simulink model "GuidanceLaw"  (R2023b)
settings: Solver=ode4  StartTime=0.0  StopTime=400  FixedStep=0.05  RelTol=1e-3
values from neighbouring files (symbols this model uses):
  APCMD_TYPE : value not decoded    [apDataDictionary.sldd]
  missionRoutePlan_struct = struct(      'validWpNum_u8', uint8(5),      'missionRoute_struct', repmat(wpDefault_struct, double(maxWpNum_u8), 1))    [initMissionRoutePlan_MC.m]
  MSSN_TYPE : value not decoded    [apDataDictionary.sldd]
  setPoint_struct = struct('lat_deg_d',double(31.200000),'lon_deg_d',double(121.500000),'alt_m_f',single(100),'yaw_deg_f',single(0))    [APTest.m]
undefined symbols (not defined in the file or in its folder): apParams
libraries: simulink x13, simulink_extras x3
(part 1 of 7)
settings Model: DataDictionary=apDataDictionary.sldd  Creator=22119  LastModifiedBy=18183
settings DataIOCC: LoggingToFile=on
settings OptimizationCC: DefaultUnderspecifiedDataType=single

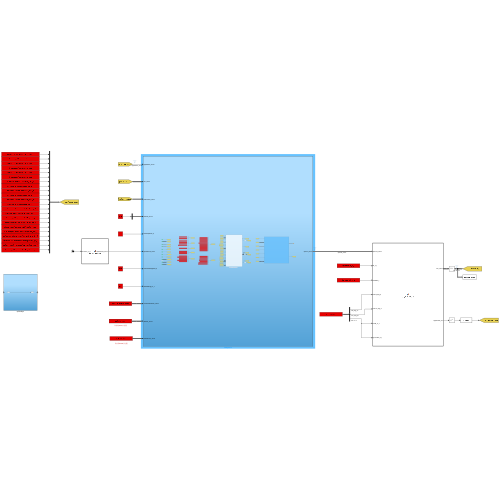
[thumbnail: Simulink's stored preview of the top-level diagram]
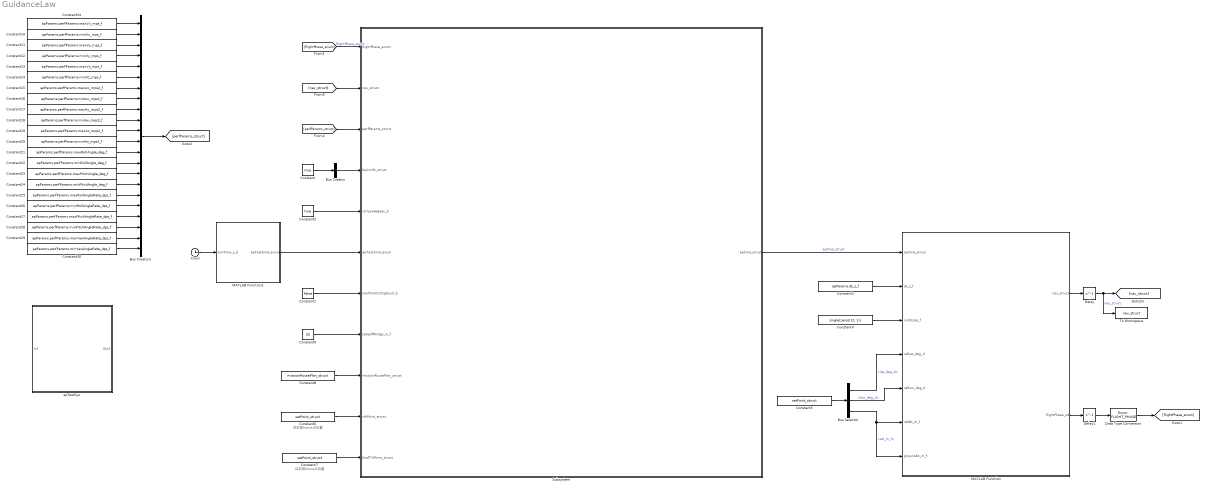
== system GuidanceLaw ==
  note: 目前是home点位置
  note: 目前用home点位置
  Bus Creator : BusCreator  Inputs=1  OutDataTypeStr=Bus: faultCaseBus
      settings: InheritFromInputs=off
  Bus Creator1 : BusCreator  Inputs=22  OutDataTypeStr=Bus: perfParamBus
      settings: InheritFromInputs=off
  Bus Selector : BusSelector  OutputSignals=lat_deg_d,lon_deg_d,alt_m_f
  Clock : Clock
  Constant : Constant  Value=true  OutDataTypeStr=boolean
  Constant1 : Constant  Value=false  OutDataTypeStr=boolean
  Constant10 : Constant  Value=apParams.perfParams.minVx_mps_f  OutDataTypeStr=single
  Constant11 : Constant  Value=apParams.perfParams.maxVy_mps_f  OutDataTypeStr=single
  Constant12 : Constant  Value=apParams.perfParams.minVy_mps_f  OutDataTypeStr=single
  Constant13 : Constant  Value=apParams.perfParams.maxVz_mps_f  OutDataTypeStr=single
  Constant14 : Constant  Value=apParams.perfParams.minVz_mps_f  OutDataTypeStr=single
  Constant15 : Constant  Value=apParams.perfParams.maxAx_mps2_f  OutDataTypeStr=single
  Constant16 : Constant  Value=apParams.perfParams.minAx_mps2_f  OutDataTypeStr=single
  Constant17 : Constant  Value=apParams.perfParams.maxAy_mps2_f  OutDataTypeStr=single
  Constant18 : Constant  Value=apParams.perfParams.minAy_mps2_f  OutDataTypeStr=single
  Constant19 : Constant  Value=apParams.perfParams.maxAz_mps2_f  OutDataTypeStr=single
  Constant2 : Constant  Value=true  OutDataTypeStr=boolean
  Constant20 : Constant  Value=apParams.perfParams.minAz_mps2_f  OutDataTypeStr=single
  Constant21 : Constant  Value=apParams.perfParams.maxRollAngle_deg_f  OutDataTypeStr=single
  Constant22 : Constant  Value=apParams.perfParams.minRollAngle_deg_f  OutDataTypeStr=single
  Constant23 : Constant  Value=apParams.perfParams.maxPitchAngle_deg_f  OutDataTypeStr=single
  Constant24 : Constant  Value=apParams.perfParams.minPitchAngle_deg_f  OutDataTypeStr=single
  Constant25 : Constant  Value=apParams.perfParams.maxRollAngleRate_dps_f  OutDataTypeStr=single
  Constant26 : Constant  Value=apParams.perfParams.minRollAngleRate_dps_f  OutDataTypeStr=single
  Constant27 : Constant  Value=apParams.perfParams.maxPitchAngleRate_dps_f  OutDataTypeStr=single
  Constant28 : Constant  Value=apParams.perfParams.minPitchAngleRate_dps_f  OutDataTypeStr=single
  Constant29 : Constant  Value=apParams.perfParams.maxYawAngleRate_dps_f  OutDataTypeStr=single
  Constant3 : Constant  Value=apParams.dt_s_f  OutDataTypeStr=single
  Constant30 : Constant  Value=apParams.perfParams.minYawAngleRate_dps_f  OutDataTypeStr=single
  Constant34 : Constant  Value=apParams.perfParams.maxVx_mps_f  OutDataTypeStr=single
  Constant4 : Constant  Value=single(zeros(12, 1))  OutDataTypeStr=single
  Constant5 : Constant  Value=setPoint_struct  OutDataTypeStr=Bus: setPointBus
  Constant6 : Constant  Value=setPoint_struct  OutDataTypeStr=Bus: setPointBus
  Constant7 : Constant  Value=setPoint_struct  OutDataTypeStr=Bus: setPointBus
  Constant8 : Constant  Value=missionRoutePlan_struct  OutDataTypeStr=Bus: missionRoutePlanBus
  Constant9 : Constant  Value=20  OutDataTypeStr=single
  Data Type Conversion : DataTypeConversion  OutDataTypeStr=Enum: FLIGHT_PHASE  SaturateOnIntegerOverflow=off  RndMeth=Floor
  Delay : Delay  DelayLength=1
  Delay1 : Delay  DelayLength=1
  MATLAB Function : MATLAB Function  TreatAsAtomicUnit=on
  MATLAB Function1 : MATLAB Function  TreatAsAtomicUnit=on
  Subsystem : Subsystem
  To Workspace : ToWorkspace  VariableName=nav_struct  SaveFormat=Timeseries  SampleTime=-1
  apTestSys : Subsystem
  wires:
  [flightPhase_enum] -> Subsystem/1(flightPhase_enum)  "flightPhase_enum"
  [perfParams_struct] -> Subsystem/3(perfParams_struct)
  Bus Creator/1 -> Subsystem/4(faultInfo_struct)
  Constant2/1 -> Subsystem/5(ctrlLawApExec_b)
  MATLAB Function1/1(apTaskCmd_enum) -> Subsystem/6(apTaskCmd_enum)
  Constant1/1 -> Subsystem/7(nonPilotCtrlSigFault_b)
  Constant9/1 -> Subsystem/8(takeoffRltHgt_m_f)
  Constant6/1 -> Subsystem/10(rthPoint_struct)
  Constant7/1 -> Subsystem/11(bwdTiltPoint_struct)
  Subsystem/1(apCmd_struct) -> MATLAB Function/1(apCmd_struct)  "apCmd_struct"
  MATLAB Function/1(nav_struct) -> Delay/1
  [nav_struct] -> Subsystem/2(nav_struct)
  Constant/1 -> Bus Creator/1
  Constant3/1 -> MATLAB Function/2(dt_s_f)
  Constant4/1 -> MATLAB Function/3(initState_f)
  Delay/1 -> To Workspace/1, [nav_struct]  "nav_struct"
  MATLAB Function/2(flightPhase_u8) -> Delay1/1
  Data Type Conversion/1 -> [flightPhase_enum]
  Delay1/1 -> Data Type Conversion/1
  Bus Creator1/1 -> [perfParams_struct]
  Constant34/1 -> Bus Creator1/1
  Constant10/1 -> Bus Creator1/2
  Constant11/1 -> Bus Creator1/3
  Constant12/1 -> Bus Creator1/4
  Constant13/1 -> Bus Creator1/5
  Constant14/1 -> Bus Creator1/6
  Constant15/1 -> Bus Creator1/7
  Constant16/1 -> Bus Creator1/8
  Constant17/1 -> Bus Creator1/9
  Constant18/1 -> Bus Creator1/10
  Constant19/1 -> Bus Creator1/11
  Constant20/1 -> Bus Creator1/12
  Constant21/1 -> Bus Creator1/13
  Constant22/1 -> Bus Creator1/14
  Constant23/1 -> Bus Creator1/15
  Constant24/1 -> Bus Creator1/16
  Constant25/1 -> Bus Creator1/17
  Constant26/1 -> Bus Creator1/18
  Constant27/1 -> Bus Creator1/19
  Constant28/1 -> Bus Creator1/20
  Clock/1 -> MATLAB Function1/1(simTime_s_d)
  Constant5/1 -> Bus Selector/1
  Bus Selector/1 -> MATLAB Function/4(refLat_deg_d)  "<lat_deg_d>"
  Bus Selector/2 -> MATLAB Function/5(refLon_deg_d)  "<lon_deg_d>"
  Bus Selector/3 -> MATLAB Function/7(groundAlt_m_f), MATLAB Function/6(refAlt_m_f)  "<alt_m_f>"
  Constant8/1 -> Subsystem/9(missionRoutePlan_struct)
  Constant29/1 -> Bus Creator1/21
  Constant30/1 -> Bus Creator1/22

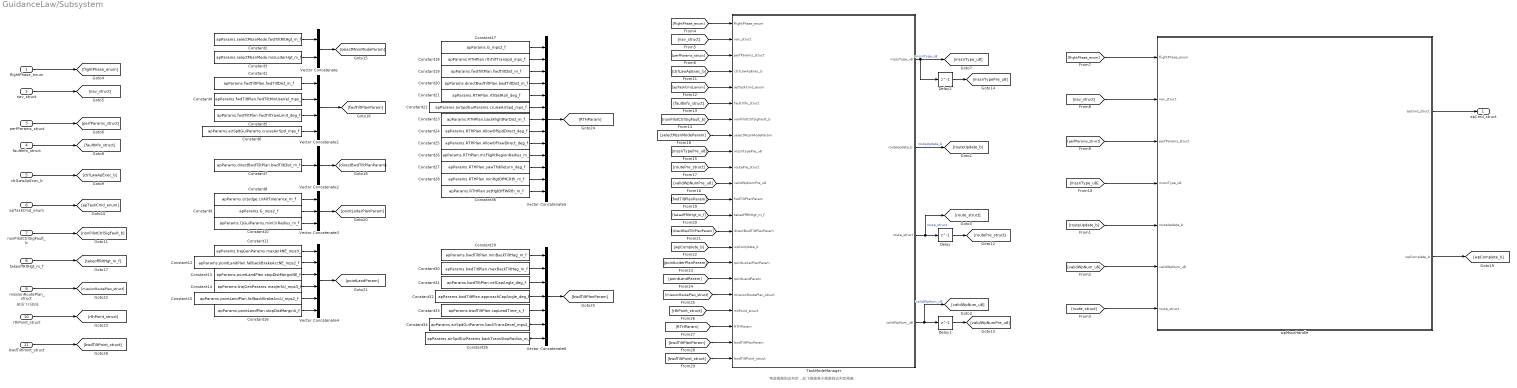
== system GuidanceLaw/Subsystem ==
  note: 航线飞行航线
  note: 考虑高度到达判定，起飞高度高于高度到达判定高度
  flightPhase_enum : Inport  OutDataTypeStr=Enum: FLIGHT_PHASE
  nav_struct : Inport  Port=2  OutDataTypeStr=Bus: apTransNavBus  BusOutputAsStruct=on
  perfParams_struct : Inport  Port=3  OutDataTypeStr=Bus: perfParamBus  BusOutputAsStruct=on
  faultInfo_struct : Inport  Port=4  OutDataTypeStr=Bus: faultCaseBus  BusOutputAsStruct=on
  ctrlLawApExec_b : Inport  Port=5  OutDataTypeStr=boolean
  apTaskCmd_enum : Inport  Port=6  OutDataTypeStr=Enum: AP_TASK_CMD
  nonPilotCtrlSigFault_b : Inport  Port=7  OutDataTypeStr=boolean
  takeoffRltHgt_m_f : Inport  Port=8  OutDataTypeStr=single
  missionRoutePlan_struct : Inport  Port=9  OutDataTypeStr=Bus: missionRoutePlanBus  BusOutputAsStruct=on
  rthPoint_struct : Inport  Port=10  OutDataTypeStr=Bus: setPointBus
  bwdTiltPoint_struct : Inport  Port=11  OutDataTypeStr=Bus: setPointBus
  Constant1 : Constant  Value=apParams.fwdTiltPlan.fwdTiltDist_m_f  OutDataTypeStr=single
  Constant10 : Constant  Value=apParams.l1GuiParams.minCirRadius_m_f  OutDataTypeStr=single
  Constant11 : Constant  Value=apParams.trajGenParams.maxJerkNE_mps3_f  OutDataTypeStr=single
  Constant12 : Constant  Value=apParams.pointLandPlan.fallbackBrakeAccNE_mps2_f  OutDataTypeStr=single
  Constant13 : Constant  Value=apParams.pointLandPlan.stopDistMarginNE_f  OutDataTypeStr=single
  Constant14 : Constant  Value=apParams.trajGenParams.maxJerkU_mps3_f  OutDataTypeStr=single
  Constant15 : Constant  Value=apParams.pointLandPlan.fallbackBrakeAccU_mps2_f  OutDataTypeStr=single
  Constant16 : Constant  Value=apParams.pointLandPlan.stopDistMarginU_f  OutDataTypeStr=single
  Constant17 : Constant  Value=apParams.G_mps2_f  OutDataTypeStr=single
  Constant18 : Constant  Value=apParams.RTHPlan.rthTiltTranSpd_mps_f  OutDataTypeStr=single
  Constant19 : Constant  Value=apParams.fwdTiltPlan.fwdTiltDist_m_f  OutDataTypeStr=single
  Constant2 : Constant  Value=apParams.selectMssnMode.fwdTiltRltHgt_m_f  OutDataTypeStr=single
  Constant20 : Constant  Value=apParams.directBwdTiltPlan.bwdTiltDist_m_f  OutDataTypeStr=single
  Constant21 : Constant  Value=apParams.RTHPlan.rthSetRoll_deg_f  OutDataTypeStr=single
  Constant22 : Constant  Value=apParams.airSpdGuiParams.cruiseAirSpd_mps_f  OutDataTypeStr=single
  Constant23 : Constant  Value=apParams.RTHPlan.backFlightFarDist_m_f  OutDataTypeStr=single
  Constant24 : Constant  Value=apParams.RTHPlan.AllowOfSpdDirect_deg_f  OutDataTypeStr=single
  Constant25 : Constant  Value=apParams.RTHPlan.AllowOfYawDirect_deg_f  OutDataTypeStr=single
  Constant26 : Constant  Value=apParams.RTHPlan.mcFlightRegionRadius_m_f  OutDataTypeStr=single
  Constant27 : Constant  Value=apParams.RTHPlan.yawThdReturn_deg_f  OutDataTypeStr=single
  Constant28 : Constant  Value=apParams.RTHPlan.minHgtOfMCRth_m_f  OutDataTypeStr=single
  Constant29 : Constant  Value=apParams.bwdTiltPlan.minBackTiltHag_m_f  OutDataTypeStr=single
  Constant3 : Constant  Value=apParams.selectMssnMode.minLoiterHgt_m_f  OutDataTypeStr=single
  Constant30 : Constant  Value=apParams.bwdTiltPlan.maxBackTiltHag_m_f  OutDataTypeStr=single
  Constant31 : Constant  Value=apParams.bwdTiltPlan.velCapAngle_deg_f  OutDataTypeStr=single
  Constant32 : Constant  Value=apParams.bwdTiltPlan.approachCapAngle_deg_f  OutDataTypeStr=single
  Constant33 : Constant  Value=apParams.bwdTiltPlan.capLeadTime_s_f  OutDataTypeStr=single
  Constant34 : Constant  Value=apParams.airSpdGuiParams.backTransDecel_mps2_f  OutDataTypeStr=single
  Constant35 : Constant  Value=apParams.airSpdGuiParams.backTransStopRadius_m_f  OutDataTypeStr=single
  Constant36 : Constant  Value=apParams.RTHPlan.setHgtOfFWRth_m_f  OutDataTypeStr=single
  Constant4 : Constant  Value=apParams.fwdTiltPlan.fwdTiltMinUseVel_mps_f  OutDataTypeStr=single
  Constant5 : Constant  Value=apParams.fwdTiltPlan.fwdTiltYawLimit_deg_f  OutDataTypeStr=single
  Constant6 : Constant  Value=apParams.airSpdGuiParams.cruiseAirSpd_mps_f  OutDataTypeStr=single
  Constant7 : Constant  Value=apParams.directBwdTiltPlan.bwdTiltDist_m_f  OutDataTypeStr=single
  Constant8 : Constant  Value=apParams.cirJudge.cirAltTolerance_m_f  OutDataTypeStr=single
  Constant9 : Constant  Value=apParams.G_mps2_f  OutDataTypeStr=single
  Delay : Delay  DelayLength=1  InitialCondition=apParams.defaultRoute_struct
  Delay1 : Delay  DelayLength=1  InitialCondition=uint8(0)
  Delay2 : Delay  DelayLength=1  InitialCondition=MSSN_TYPE.IDLE
  TaskModeManager : Stateflow chart  TreatAsAtomicUnit=on
  Vector Concatenate : Concatenate
  Vector Concatenate1 : Concatenate  NumInputs=4
  Vector Concatenate2 : Concatenate  NumInputs=1
  Vector Concatenate3 : Concatenate  NumInputs=3
  Vector Concatenate4 : Concatenate  NumInputs=6
  Vector Concatenate5 : Concatenate  NumInputs=13
  Vector Concatenate6 : Concatenate  NumInputs=7
  wpMssnHandle : Subsystem
  apCmd_struct : Outport  OutDataTypeStr=Bus: apCmdBus
  wires:
  TaskModeManager/2(routeUpdate_b) -> [routeUpdate_b]  "routeUpdate_b"
  [perfParams_struct] -> wpMssnHandle/3(perfParams_struct)
  Constant30/1 -> Vector Concatenate6/2
  Constant19/1 -> Vector Concatenate5/3
  Vector Concatenate1/1 -> [fwdTiltPlanParam]
  [flightPhase_enum] -> wpMssnHandle/1(flightPhase_enum)
  [ctrlLawApExec_b] -> TaskModeManager/4(ctrlLawApExec_b)
  Constant17/1 -> Vector Concatenate5/1
  [nav_struct] -> TaskModeManager/2(nav_struct)
  Delay2/1 -> [mssnTypePre_u8]
  Vector Concatenate4/1 -> [pointLandParam]
  Constant32/1 -> Vector Concatenate6/4
  [routeUpdate_b] -> wpMssnHandle/5(routeUpdate_b)
  [rthPoint_struct] -> TaskModeManager/19(rthPoint_struct)
  [nonPilotCtrlSigFault_b] -> TaskModeManager/7(nonPilotCtrlSigFault_b)
  [mssnType_u8] -> wpMssnHandle/4(mssnType_u8)
  flightPhase_enum/1 -> [flightPhase_enum]
  [pointLandParam] -> TaskModeManager/17(pointLandParam)
  Constant25/1 -> Vector Concatenate5/9
  faultInfo_struct/1 -> [faultInfo_struct]
  [takeoffRltHgt_m_f] -> TaskModeManager/13(takeoffRltHgt_m_f)
  [validWpNumPre_u8] -> TaskModeManager/11(validWpNumPre_u8)
  Vector Concatenate6/1 -> [bwdTiltPlanParam]
  [faultInfo_struct] -> TaskModeManager/6(faultInfo_struct)
  perfParams_struct/1 -> [perfParams_struct]
  Constant21/1 -> Vector Concatenate5/5
  Constant29/1 -> Vector Concatenate6/1
  ctrlLawApExec_b/1 -> [ctrlLawApExec_b]
  [nav_struct] -> wpMssnHandle/2(nav_struct)
  Vector Concatenate5/1 -> [RTHParam]
  [routePre_struct] -> TaskModeManager/10(routePre_struct)
  Constant33/1 -> Vector Concatenate6/5
  Constant18/1 -> Vector Concatenate5/2
  Constant20/1 -> Vector Concatenate5/4
  [missionRoutePlan_struct] -> TaskModeManager/18(missionRoutePlan_struct)
  Constant22/1 -> Vector Concatenate5/6
  TaskModeManager/1(mssnType_u8) -> Delay2/1, [mssnType_u8]  "mssnType_u8"
  [fwdTiltPlanParam] -> TaskModeManager/12(fwdTiltPlanParam)
  [bwdTiltPoint_struct] -> TaskModeManager/22(bwdTiltPoint_struct)
  Constant11/1 -> Vector Concatenate4/1
  apTaskCmd_enum/1 -> [apTaskCmd_enum]
  [flightPhase_enum] -> TaskModeManager/1(flightPhase_enum)
  Constant4/1 -> Vector Concatenate1/2
  [pointLoiterPlanParam] -> TaskModeManager/16(pointLoiterPlanParam)
  Constant1/1 -> Vector Concatenate1/1
  [RTHParam] -> TaskModeManager/20(RTHParam)
  [perfParams_struct] -> TaskModeManager/3(perfParams_struct)
  TaskModeManager/3(route_struct) -> [route_struct], Delay/1  "route_struct"
  Constant12/1 -> Vector Concatenate4/2
  [wpComplete_b] -> TaskModeManager/15(wpComplete_b)
  Constant15/1 -> Vector Concatenate4/5
  Vector Concatenate3/1 -> [pointLoiterPlanParam]
  [directBwdTiltPlanParam] -> TaskModeManager/14(directBwdTiltPlanParam)
  Constant23/1 -> Vector Concatenate5/7
  Constant27/1 -> Vector Concatenate5/11
  Constant14/1 -> Vector Concatenate4/4
  Constant8/1 -> Vector Concatenate3/1
  Vector Concatenate2/1 -> [directBwdTiltPlanParam]
  Constant3/1 -> Vector Concatenate/2
  [route_struct] -> wpMssnHandle/7(route_struct)
  Delay1/1 -> [validWpNumPre_u8]
  [apTaskCmd_enum] -> TaskModeManager/5(apTaskCmd_enum)
  nonPilotCtrlSigFault_b/1 -> [nonPilotCtrlSigFault_b]
  wpMssnHandle/1(apCmd_struct) -> apCmd_struct/1
  Constant2/1 -> Vector Concatenate/1
  [validWpNum_u8] -> wpMssnHandle/6(validWpNum_u8)
  Constant28/1 -> Vector Concatenate5/12
  Constant26/1 -> Vector Concatenate5/10
  Constant13/1 -> Vector Concatenate4/3
  Constant10/1 -> Vector Concatenate3/3
  Constant24/1 -> Vector Concatenate5/8
  rthPoint_struct/1 -> [rthPoint_struct]
  TaskModeManager/4(validWpNum_u8) -> [validWpNum_u8], Delay1/1  "validWpNum_u8"
  nav_struct/1 -> [nav_struct]
  Constant6/1 -> Vector Concatenate1/4
  Vector Concatenate/1 -> [selectMssnModeParam]
  Constant5/1 -> Vector Concatenate1/3
  Constant31/1 -> Vector Concatenate6/3
  [selectMssnModeParam] -> TaskModeManager/8(selectMssnModeParam)
  bwdTiltPoint_struct/1 -> [bwdTiltPoint_struct]
  missionRoutePlan_struct/1 -> [missionRoutePlan_struct]
  [mssnTypePre_u8] -> TaskModeManager/9(mssnTypePre_u8)
  takeoffRltHgt_m_f/1 -> [takeoffRltHgt_m_f]
  [bwdTiltPlanParam] -> TaskModeManager/21(bwdTiltPlanParam)
  Constant16/1 -> Vector Concatenate4/6
  Constant7/1 -> Vector Concatenate2/1
  Constant34/1 -> Vector Concatenate6/6
  Delay/1 -> [routePre_struct]
  Constant9/1 -> Vector Concatenate3/2
  wpMssnHandle/2(wpComplete_b) -> [wpComplete_b]
  Constant35/1 -> Vector Concatenate6/7
  Constant36/1 -> Vector Concatenate5/13

== system GuidanceLaw/apTestSys ==
  In1 : Inport
  Out1 : Outport
  wires:
  In1/1 -> Out1/1

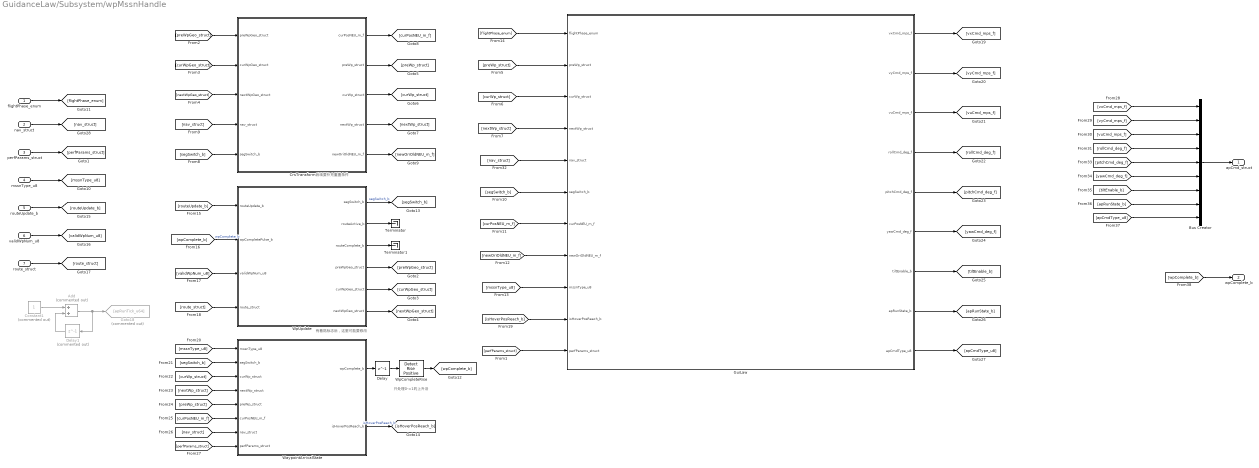
== system GuidanceLaw/Subsystem/wpMssnHandle ==
  note: 后续要补充重置条件
  note: 只处理0->1的上升沿
  note: 有着陆标志后，这里可能要修改
  flightPhase_enum : Inport
  nav_struct : Inport  Port=2
  perfParams_struct : Inport  Port=3
  mssnType_u8 : Inport  Port=4
  routeUpdate_b : Inport  Port=5
  validWpNum_u8 : Inport  Port=6
  route_struct : Inport  Port=7  PortDimensions=[30,1]  BusOutputAsStruct=on
  Add : Sum  Commented=on  OutDataTypeStr=uint64  AccumDataTypeStr=uint64
  Bus Creator : BusCreator  Inputs=9  OutDataTypeStr=Bus: apCmdBus
      settings: InheritFromInputs=off
  Constant1 : Constant  Commented=on  OutDataTypeStr=uint64
  CrsTransform : Subsystem
  Delay : Delay  DelayLength=1  InitialCondition=false
  Delay1 : Delay  Commented=on  DelayLength=1  InitialCondition=uint64(0)
  Goto18 : Goto  Commented=on  GotoTag=apRunTick_u64
  GuiLaw : Subsystem
  Terminator : Terminator
  Terminator1 : Terminator
  WaypointArrivalState : Subsystem
  WpCompleteRise : simulink/Logic and Bit Operations/Detect Rise Positive  vinit=0  OutDataTypeStr=boolean
  WpUpdate : Subsystem
  apCmd_struct : Outport  OutDataTypeStr=Bus: apCmdBus
  wpComplete_b : Outport  Port=2
  wires:
  [preWp_struct] -> WaypointArrivalState/5(preWp_struct)
  mssnType_u8/1 -> [mssnType_u8]
  GuiLaw/6(yawCmd_deg_f) -> [yawCmd_deg_f]
  WpUpdate/6(nextWpGeo_struct) -> [nextWpGeo_struct]
  [newOriOldNEU_m_f] -> GuiLaw/8(newOriOldNEU_m_f)
  [segSwitch_b] -> WaypointArrivalState/2(segSwitch_b)
  WpUpdate/5(curWpGeo_struct) -> [curWpGeo_struct]
  [isHoverPosReach_b] -> GuiLaw/10(isHoverPosReach_b)
  WpUpdate/4(preWpGeo_struct) -> [preWpGeo_struct]
  GuiLaw/7(tiltEnable_b) -> [tiltEnable_b]
  WaypointArrivalState/1(wpComplete_b) -> Delay/1
  [flightPhase_enum] -> GuiLaw/1(flightPhase_enum)
  [segSwitch_b] -> GuiLaw/6(segSwitch_b)
  [segSwitch_b] -> CrsTransform/5(segSwitch_b)
  WaypointArrivalState/2(isHoverPosReach_b) -> [isHoverPosReach_b]  "isHoverPosReach_b"
  nav_struct/1 -> [nav_struct]
  WpUpdate/1(segSwitch_b) -> [segSwitch_b]  "segSwitch_b"
  WpUpdate/2(routeActive_b) -> Terminator/1
  [curWp_struct] -> WaypointArrivalState/3(curWp_struct)
  GuiLaw/3(vuCmd_mps_f) -> [vuCmd_mps_f]
  Delay/1 -> WpCompleteRise/1
  [mssnType_u8] -> GuiLaw/9(mssnType_u8)
  [nextWp_struct] -> WaypointArrivalState/4(nextWp_struct)
  CrsTransform/5(newOriOldNEU_m_f) -> [newOriOldNEU_m_f]
  CrsTransform/1(curPosNEU_m_f) -> [curPosNEU_m_f]
  GuiLaw/4(rollCmd_deg_f) -> [rollCmd_deg_f]
  Add/1 -> Delay1/1, Goto18/1
  [preWp_struct] -> GuiLaw/2(preWp_struct)
  [route_struct] -> WpUpdate/4(route_struct)
  Delay1/1 -> Add/2
  [mssnType_u8] -> WaypointArrivalState/1(mssnType_u8)
  [nav_struct] -> WaypointArrivalState/7(nav_struct)
  [perfParams_struct] -> GuiLaw/11(perfParams_struct)
  validWpNum_u8/1 -> [validWpNum_u8]
  [curWpGeo_struct] -> CrsTransform/2(curWpGeo_struct)
  CrsTransform/4(nextWp_struct) -> [nextWp_struct]
  route_struct/1 -> [route_struct]
  [curPosNEU_m_f] -> WaypointArrivalState/6(curPosNEU_m_f)
  GuiLaw/9(apCmdType_u8) -> [apCmdType_u8]
  WpUpdate/3(routeComplete_b) -> Terminator1/1
  flightPhase_enum/1 -> [flightPhase_enum]
  GuiLaw/5(pitchCmd_deg_f) -> [pitchCmd_deg_f]
  [curPosNEU_m_f] -> GuiLaw/7(curPosNEU_m_f)
  Constant1/1 -> Add/1
  GuiLaw/8(apRunState_b) -> [apRunState_b]
  GuiLaw/2(vyCmd_mps_f) -> [vyCmd_mps_f]
  [perfParams_struct] -> WaypointArrivalState/8(perfParams_struct)
  perfParams_struct/1 -> [perfParams_struct]
  [routeUpdate_b] -> WpUpdate/1(routeUpdate_b)
  CrsTransform/3(curWp_struct) -> [curWp_struct]
  [nextWpGeo_struct] -> CrsTransform/3(nextWpGeo_struct)
  routeUpdate_b/1 -> [routeUpdate_b]
  [nav_struct] -> CrsTransform/4(nav_struct)
  CrsTransform/2(preWp_struct) -> [preWp_struct]
  [preWpGeo_struct] -> CrsTransform/1(preWpGeo_struct)
  [wpComplete_b] -> WpUpdate/2(wpCompletePulse_b)  "wpComplete_b"
  [nav_struct] -> GuiLaw/5(nav_struct)
  [curWp_struct] -> GuiLaw/3(curWp_struct)
  [nextWp_struct] -> GuiLaw/4(nextWp_struct)
  [validWpNum_u8] -> WpUpdate/3(validWpNum_u8)
  GuiLaw/1(vxCmd_mps_f) -> [vxCmd_mps_f]
  [vxCmd_mps_f] -> Bus Creator/1
  [vyCmd_mps_f] -> Bus Creator/2
  [vuCmd_mps_f] -> Bus Creator/3
  [rollCmd_deg_f] -> Bus Creator/4
  [pitchCmd_deg_f] -> Bus Creator/5
  [yawCmd_deg_f] -> Bus Creator/6
  [tiltEnable_b] -> Bus Creator/7
  [apRunState_b] -> Bus Creator/8
  [apCmdType_u8] -> Bus Creator/9
  Bus Creator/1 -> apCmd_struct/1
  [wpComplete_b] -> wpComplete_b/1
  WpCompleteRise/1 -> [wpComplete_b]

== system GuidanceLaw/Subsystem/wpMssnHandle/CrsTransform ==
  preWpGeo_struct : Inport
  curWpGeo_struct : Inport  Port=2
  nextWpGeo_struct : Inport  Port=3
  nav_struct : Inport  Port=4
  segSwitch_b : Inport  Port=5
  Bus Creator : BusCreator  Inputs=11  OutDataTypeStr=Bus: localNEUWpBus
      settings: InheritFromInputs=off
  Bus Creator1 : BusCreator  Inputs=11  OutDataTypeStr=Bus: localNEUWpBus
      settings: InheritFromInputs=off
  Bus Creator2 : BusCreator  Inputs=11  OutDataTypeStr=Bus: localNEUWpBus
      settings: InheritFromInputs=off
  Bus Selector : BusSelector  OutputSignals=wpType_u8,spd_mps_f,radius_m_f,fastWp_b,yawType_u8,yaw_deg_f,timeOrCount_u16,arrivalCond_u8
  Bus Selector1 : BusSelector  OutputSignals=wpType_u8,spd_mps_f,radius_m_f,fastWp_b,yawType_u8,yaw_deg_f,timeOrCount_u16,arrivalCond_u8
  Bus Selector2 : BusSelector  OutputSignals=wpType_u8,spd_mps_f,radius_m_f,fastWp_b,yawType_u8,yaw_deg_f,timeOrCount_u16,arrivalCond_u8
  Demux : Demux  Outputs=3
  Demux1 : Demux  Outputs=3
  Demux2 : Demux  Outputs=3
  geoToLocalNEU : MATLAB Function  TreatAsAtomicUnit=on
  curPosNEU_m_f : Outport
  preWp_struct : Outport  Port=2
  curWp_struct : Outport  Port=3
  nextWp_struct : Outport  Port=4
  newOriOldNEU_m_f : Outport  Port=5
  wires:
  preWpGeo_struct/1 -> [preWpGeo_struct]
  curWpGeo_struct/1 -> [curWpGeo_struct]
  nextWpGeo_struct/1 -> [nextWpGeo_struct]
  [preWpGeo_struct] -> geoToLocalNEU/2(preWpGeo_struct)
  [curWpGeo_struct] -> geoToLocalNEU/3(curWpGeo_struct)
  [nextWpGeo_struct] -> geoToLocalNEU/4(nextWpGeo_struct)
  nav_struct/1 -> [nav_struct]
  [nav_struct] -> geoToLocalNEU/1(curGeo_struct)
  [segSwitch_b] -> geoToLocalNEU/5(segSwitch_b)
  segSwitch_b/1 -> [segSwitch_b]
  geoToLocalNEU/1(curPosNEU_m_f) -> curPosNEU_m_f/1
  geoToLocalNEU/5(newOriOldNEU_m_f) -> newOriOldNEU_m_f/1
  [preWpGeo_struct] -> Bus Selector/1
  Bus Selector/1 -> Bus Creator/1  "<wpType_u8>"
  Bus Selector/2 -> Bus Creator/5  "<spd_mps_f>"
  Bus Selector/3 -> Bus Creator/6  "<radius_m_f>"
  Bus Selector/4 -> Bus Creator/7  "<fastWp_b>"
  Bus Selector/5 -> Bus Creator/8  "<yawType_u8>"
  Bus Selector/6 -> Bus Creator/9  "<yaw_deg_f>"
  geoToLocalNEU/2(preWpNEU_m_f) -> [preWpNEU_m_f]
  geoToLocalNEU/3(curWpNEU_m_f) -> [curWpNEU_m_f]
  geoToLocalNEU/4(nextWpNEU_m_f) -> [nextWpNEU_m_f]
  Bus Creator/1 -> preWp_struct/1
  Demux/1 -> Bus Creator/2
  Demux/2 -> Bus Creator/3
  Demux/3 -> Bus Creator/4
  [preWpNEU_m_f] -> Demux/1
  Demux1/2 -> Bus Creator1/3
  Demux1/1 -> Bus Creator1/2
  Bus Creator1/1 -> curWp_struct/1
  [curWpGeo_struct] -> Bus Selector1/1
  Bus Selector1/2 -> Bus Creator1/5  "<spd_mps_f>"
  Bus Selector1/3 -> Bus Creator1/6  "<radius_m_f>"
  Bus Selector1/6 -> Bus Creator1/9  "<yaw_deg_f>"
  Bus Selector1/5 -> Bus Creator1/8  "<yawType_u8>"
  Bus Selector1/4 -> Bus Creator1/7  "<fastWp_b>"
  Bus Selector1/1 -> Bus Creator1/1  "<wpType_u8>"
  Demux1/3 -> Bus Creator1/4
  [curWpNEU_m_f] -> Demux1/1
  Bus Selector2/1 -> Bus Creator2/1  "<wpType_u8>"
  Demux2/3 -> Bus Creator2/4
  [nextWpNEU_m_f] -> Demux2/1
  Bus Selector2/4 -> Bus Creator2/7  "<fastWp_b>"
  Bus Selector2/6 -> Bus Creator2/9  "<yaw_deg_f>"
  Bus Selector2/3 -> Bus Creator2/6  "<radius_m_f>"
  Bus Selector2/2 -> Bus Creator2/5  "<spd_mps_f>"
  Demux2/2 -> Bus Creator2/3
  Bus Selector2/5 -> Bus Creator2/8  "<yawType_u8>"
  [nextWpGeo_struct] -> Bus Selector2/1
  Demux2/1 -> Bus Creator2/2
  Bus Creator2/1 -> nextWp_struct/1
  Bus Selector/7 -> Bus Creator/10  "<timeOrCount_u16>"
  Bus Selector/8 -> Bus Creator/11  "<arrivalCond_u8>"
  Bus Selector1/7 -> Bus Creator1/10  "<timeOrCount_u16>"
  Bus Selector1/8 -> Bus Creator1/11  "<arrivalCond_u8>"
  Bus Selector2/7 -> Bus Creator2/10  "<timeOrCount_u16>"
  Bus Selector2/8 -> Bus Creator2/11  "<arrivalCond_u8>"

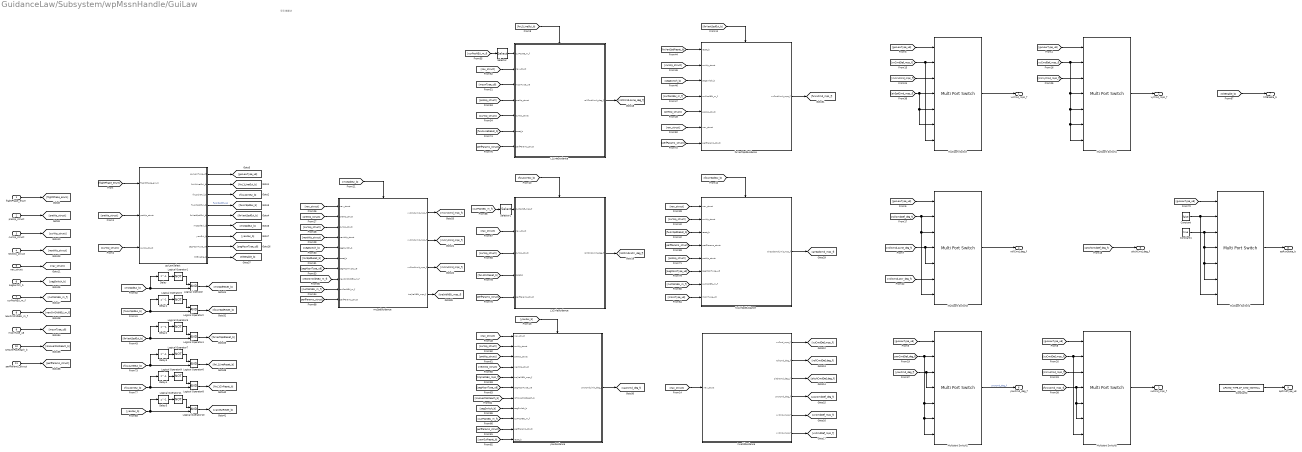
== system GuidanceLaw/Subsystem/wpMssnHandle/GuiLaw ==
  note: 导引律算法
  flightPhase_enum : Inport
  preWp_struct : Inport  Port=2
  curWp_struct : Inport  Port=3
  nextWp_struct : Inport  Port=4
  nav_struct : Inport  Port=5
  segSwitch_b : Inport  Port=6
  curPosNEU_m_f : Inport  Port=7
  newOriOldNEU_m_f : Inport  Port=8
  mssnType_u8 : Inport  Port=9
  isHoverPosReach_b : Inport  Port=10
  perfParams_struct : Inport  Port=11
  Constant : Constant  Value=false  OutDataTypeStr=boolean
  Constant1 : Constant  Value=true  OutDataTypeStr=boolean
  Constant2 : Constant  Value=APCMD_TYPE.AP_CMD_NORMAL  VectorParams1D=off  OutDataTypeStr=Enum: APCMD_TYPE
  Delay{,1..5} (6 alike) : Delay  DelayLength=1  InitialCondition=false
  L1CirleGuidance : Subsystem
  L1LineGuidance : Subsystem
  Logical Operator{,2,4,6,8,10} (6 alike) : Logic  AllPortsSameDT=off  OutDataTypeStr=boolean
  Logical Operator{1,3,5,7,9,11} (6 alike) : Logic  Operator=NOT  AllPortsSameDT=off  OutDataTypeStr=boolean
  Multiport Switch{,1..5} (6 alike) : MultiPortSwitch  DataPortOrder=Zero-based contiguous  Inputs=5  DataPortForDefault=Additional data port  DiagnosticForDefault=None  zeroidx=on  SaturateOnIntegerOverflow=off  InputSameDT=off
  Selector : Selector  InputPortWidth=3  IndexOptions=Index vector (dialog)  Indices=[1 2]  OutputSizes=1
  Selector1 : Selector  InputPortWidth=3  IndexOptions=Index vector (dialog)  Indices=[1 2]  OutputSizes=1
  fwAirSpdGuidance : Subsystem
  fwVertSpdGuidance : Subsystem
  guiLawSelect : Subsystem
  invaildGuidance : Subsystem
  mcSpdGuidance : Subsystem
  yawGuidance : Subsystem
  vxCmd_mps_f : Outport
  vyCmd_mps_f : Outport  Port=2
  vuCmd_mps_f : Outport  Port=3
  rollCmd_deg_f : Outport  Port=4
  pitchCmd_deg_f : Outport  Port=5
  yawCmd_deg_f : Outport  Port=6
  tiltEnable_b : Outport  Port=7
  apRunState_b : Outport  Port=8
  apCmdType_u8 : Outport  Port=9
  wires:
  [preWp_struct] -> fwVertSpdGuidance/5(preWp_struct)
  [mcSpdGui_b] -> mcSpdGuidance/Enable
  [yawCmd_deg_f] -> Multiport Switch2/4, Multiport Switch2/3
  [segMssnType_u8] -> mcSpdGuidance/7(segMssnType_u8)
  [preWp_struct] -> L1LineGuidance/4(preWp_struct)
  [rollCmdL1Line_deg_f] -> Multiport Switch3/5, Multiport Switch3/4
  guiLawSelect/7(yawGui_b) -> [yawGui_b]
  [segSwitch_b] -> fwVertSpdGuidance/3(segSwitch_b)
  [curPosNEU_m_f] -> Selector/1
  Logical Operator/1 -> [mcSpdReset_b]
  [nav_struct] -> yawGuidance/1(nav_struct)
  [curPosNEU_m_f] -> fwVertSpdGuidance/4(curPosNEU_m_f)
  [segSwitch_b] -> yawGuidance/8(segSwitch_b)
  [fwL1CirGui_b] -> L1CirleGuidance/Enable
  [rollCmdDef_deg_f] -> Multiport Switch3/3, Multiport Switch3/7, Multiport Switch3/2
  [curPosNEU_m_f] -> Selector1/1
  [fwAirSpdGui_b] -> fwAirSpdGuidance/Enable
  [guiLawType_u8] -> Multiport Switch2/1
  [preWp_struct] -> guiLawSelect/2(preWp_struct)
  [airSpdCmd_mps_f] -> Multiport Switch/6, Multiport Switch/5, Multiport Switch/4
  guiLawSelect/1(guiLawType_u8) -> [guiLawType_u8]
  [fwVertSpdGui_b] -> Delay2/1, Logical Operator4/2
  [curWp_struct] -> fwAirSpdGuidance/2(curWp_struct)
  Delay2/1 -> Logical Operator5/1
  mcSpdGuidance/1(vxCmdLimit_mps_f) -> [mcVxCmd_mps_f]
  Multiport Switch3/1 -> rollCmd_deg_f/1
  mcSpdGuidance/4(trajVelNEU_mps_f) -> [trajVelNEU_mps_f]
  [vxCmdDef_mps_f] -> Multiport Switch/7, Multiport Switch/2
  [guiLawType_u8] -> Multiport Switch3/1
  [guiLawType_u8] -> Multiport Switch/1
  [guiLawType_u8] -> Multiport Switch1/1
  [flightPhase_enum] -> guiLawSelect/1(flightPhase_enum)
  guiLawSelect/4(fwAirSpdGui_b) -> [fwAirSpdGui_b]  "fwAirSpdGui_b"
  [mcSpdGui_b] -> Delay/1, Logical Operator/2
  segSwitch_b/1 -> [segSwitch_b]
  curWp_struct/1 -> [curWp_struct]
  Multiport Switch5/1 -> vuCmd_mps_f/1
  [trajVelNEU_mps_f] -> yawGuidance/5(trajVelNEU_mps_f)
  mssnType_u8/1 -> [mssnType_u8]
  Logical Operator5/1 -> Logical Operator4/1
  [nav_struct] -> fwAirSpdGuidance/1(nav_struct)
  guiLawSelect/5(fwVertSpdGui_b) -> [fwVertSpdGui_b]
  [nav_struct] -> fwVertSpdGuidance/6(nav_struct)
  Delay1/1 -> Logical Operator3/1
  [segMssnType_u8] -> yawGuidance/6(segMssnType_u8)
  [fwAirSpdReset_b] -> fwAirSpdGuidance/3(reset_b)
  [nav_struct] -> L1LineGuidance/2(nav_struct)
  [fwVertSpdGui_b] -> fwVertSpdGuidance/Enable
  [mcVuCmd_mps_f] -> Multiport Switch5/3
  [mssnType_u8] -> L1LineGuidance/3(mssnType_u8)
  [mcVxCmd_mps_f] -> Multiport Switch/3
  yawGuidance/1(yawCmdLimit_deg_f) -> [yawCmd_deg_f]
  [isHoverPosReach_b] -> yawGuidance/7(isHoverPosReach_b)
  [curWp_struct] -> L1CirleGuidance/3(curWp_struct)
  guiLawSelect/3(fwL1CirGui_b) -> [fwL1CirGui_b]
  [newOriOldNEU_m_f] -> mcSpdGuidance/8(newOriOldNEU_m_f)
  invaildGuidance/1(vuCmd_mps_f) -> [vuCmdDef_mps_f]
  guiLawSelect/6(mcSpdGui_b) -> [mcSpdGui_b]
  [curWp_struct] -> yawGuidance/2(curWp_struct)
  [nextWp_struct] -> yawGuidance/4(nextWp_struct)
  [curWp_struct] -> fwVertSpdGuidance/2(curWp_struct)
  [preWp_struct] -> yawGuidance/3(preWp_struct)
  [rollCmdL1Cir_deg_f] -> Multiport Switch3/6
  Selector1/1 -> L1CirleGuidance/1(curPosNE_mps_f)
  [fwL1LineGui_b] -> L1LineGuidance/Enable
  [curWp_struct] -> guiLawSelect/3(curWp_struct)
  isHoverPosReach_b/1 -> [isHoverPosReach_b]
  [mcVyCmd_mps_f] -> Multiport Switch1/3
  guiLawSelect/2(fwL1LineGui_b) -> [fwL1LineGui_b]
  Selector/1 -> L1LineGuidance/1(curPosNE_m_f)
  preWp_struct/1 -> [preWp_struct]
  [nav_struct] -> L1CirleGuidance/2(nav_struct)
  invaildGuidance/4(yawCmd_deg_f) -> [yawCmdDef_deg_f]
  [yawGui_b] -> yawGuidance/Enable
  L1CirleGuidance/1(rollCmdLimit_deg_f) -> [rollCmdL1Cir_deg_f]
  [guiLawType_u8] -> Multiport Switch5/1
  nav_struct/1 -> [nav_struct]
  invaildGuidance/6(vxCmd_mps_f) -> [vxCmdDef_mps_f]
  [vyCmdDef_mps_f] -> Multiport Switch1/4, Multiport Switch1/6, Multiport Switch1/7, Multiport Switch1/5, Multiport Switch1/2
  Logical Operator4/1 -> [fwVertSpdReset_b]
  Logical Operator3/1 -> Logical Operator2/1
  [yawCmdDef_deg_f] -> Multiport Switch2/5, Multiport Switch2/6, Multiport Switch2/7, Multiport Switch2/2
  [nav_struct] -> invaildGuidance/1(nav_struct)
  mcSpdGuidance/3(vuCmdLimit_mps_f) -> [mcVuCmd_mps_f]
  Multiport Switch/1 -> vxCmd_mps_f/1
  fwAirSpdGuidance/1(airSpdCmdLimit_mps_f) -> [airSpdCmd_mps_f]
  Multiport Switch1/1 -> vyCmd_mps_f/1
  [pitchCmdDef_deg_f] -> pitchCmd_deg_f/1
  newOriOldNEU_m_f/1 -> [newOriOldNEU_m_f]
  Multiport Switch2/1 -> yawCmd_deg_f/1  "yawCmd_deg_f"
  L1LineGuidance/1(rollCmdLimit_deg_f) -> [rollCmdL1Line_deg_f]
  [vuCmdDef_mps_f] -> Multiport Switch5/7, Multiport Switch5/2
  invaildGuidance/2(rollCmd_deg_f) -> [rollCmdDef_deg_f]
  Logical Operator1/1 -> Logical Operator/1
  Delay/1 -> Logical Operator1/1
  [fwAirSpdGui_b] -> Delay1/1, Logical Operator2/2
  [preWp_struct] -> mcSpdGuidance/2(preWp_struct)
  invaildGuidance/5(vyCmd_mps_f) -> [vyCmdDef_mps_f]
  curPosNEU_m_f/1 -> [curPosNEU_m_f]
  [mcSpdReset_b] -> mcSpdGuidance/6(reset_b)
  [segSwitch_b] -> mcSpdGuidance/5(segSwitch_b)
  [curWp_struct] -> mcSpdGuidance/3(curWp_struct)
  [nav_struct] -> mcSpdGuidance/1(nav_struct)
  fwVertSpdGuidance/1(vuCmdLimit_mps_f) -> [fwVuCmd_mps_f]
  [fwVuCmd_mps_f] -> Multiport Switch5/6, Multiport Switch5/5, Multiport Switch5/4
  mcSpdGuidance/2(vyCmdLimit_mps_f) -> [mcVyCmd_mps_f]
  Logical Operator2/1 -> [fwAirSpdReset_b]
  flightPhase_enum/1 -> [flightPhase_enum]
  nextWp_struct/1 -> [nextWp_struct]
  invaildGuidance/3(pitchCmd_deg_f) -> [pitchCmdDef_deg_f]
  [curPosNEU_m_f] -> mcSpdGuidance/9(curPosNEU_m_f)
  [fwVertSpdReset_b] -> fwVertSpdGuidance/1(reset_b)
  [nextWp_struct] -> mcSpdGuidance/4(nextWp_struct)
  guiLawSelect/8(segMssnType_u8) -> [segMssnType_u8]
  [curWp_struct] -> L1LineGuidance/5(curWp_struct)
  [curPosNEU_m_f] -> yawGuidance/9(curPosNEU_m_f)
  guiLawSelect/9(tiltEnable_b) -> [tiltEnable_b]
  [tiltEnable_b] -> tiltEnable_b/1
  perfParams_struct/1 -> [perfParams_struct]
  [perfParams_struct] -> mcSpdGuidance/10(perfParams_struct)
  [perfParams_struct] -> fwAirSpdGuidance/4(perfParams_struct)
  Multiport Switch4/1 -> apRunState_b/1
  [guiLawType_u8] -> Multiport Switch4/1
  Constant/1 -> Multiport Switch4/7, Multiport Switch4/2
  Constant1/1 -> Multiport Switch4/6, Multiport Switch4/5, Multiport Switch4/4, Multiport Switch4/3
  [preWp_struct] -> fwAirSpdGuidance/5(preWp_struct)
  [perfParams_struct] -> fwVertSpdGuidance/7(perfParams_struct)
  [fwL1LineGui_b] -> Delay3/1, Logical Operator6/2
  Logical Operator7/1 -> Logical Operator6/1
  Logical Operator6/1 -> [fwL1LineReset_b]
  Delay3/1 -> Logical Operator7/1
  [fwL1LineReset_b] -> L1LineGuidance/6(reset_b)
  [perfParams_struct] -> L1LineGuidance/7(perfParams_struct)
  [perfParams_struct] -> L1CirleGuidance/5(perfParams_struct)
  Logical Operator8/1 -> [fwL1CirReset_b]
  Logical Operator9/1 -> Logical Operator8/1
  [fwL1CirGui_b] -> Delay4/1, Logical Operator8/2
  Delay4/1 -> Logical Operator9/1
  [fwL1CirReset_b] -> L1CirleGuidance/4(reset_b)
  [segMssnType_u8] -> fwAirSpdGuidance/6(segMssnType_u8)
  [curPosNEU_m_f] -> fwAirSpdGuidance/7(curPosNEU_m_f)
  Constant2/1 -> apCmdType_u8/1
  [perfParams_struct] -> yawGuidance/10(perfParams_struct)
  [yawGuiReset_b] -> yawGuidance/11(reset_b)
  Delay5/1 -> Logical Operator11/1
  [yawGui_b] -> Logical Operator10/2, Delay5/1
  Logical Operator11/1 -> Logical Operator10/1
  Logical Operator10/1 -> [yawGuiReset_b]
  [mssnType_u8] -> fwAirSpdGuidance/8(mssnType_u8)

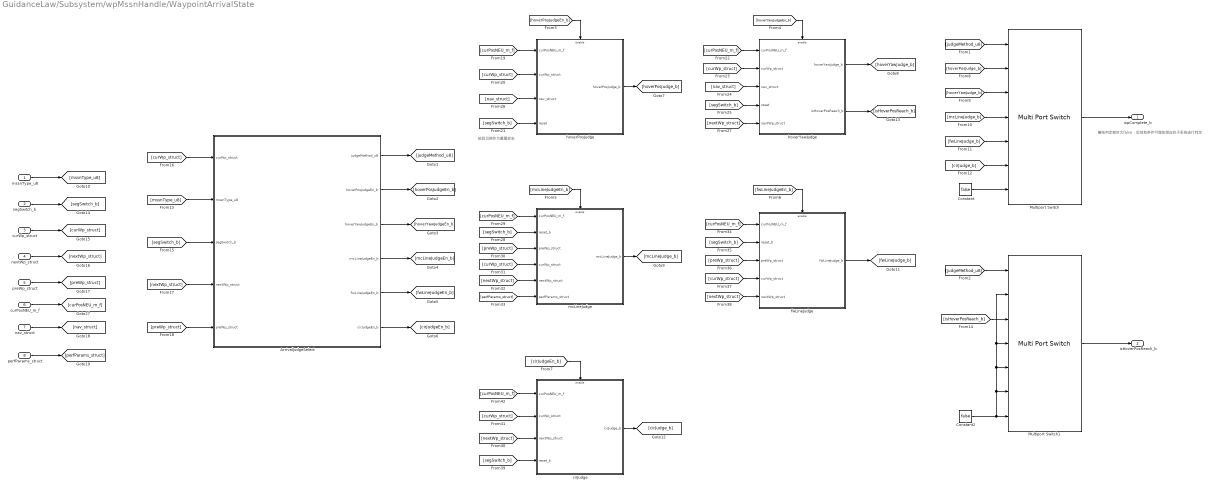
== system GuidanceLaw/Subsystem/wpMssnHandle/WaypointArrivalState ==
  note: 航段切换作为重置标志
  note: 着陆判定暂时为false，后续有条件可增加相应的子系统进行判定
  mssnType_u8 : Inport
  segSwitch_b : Inport  Port=2
  curWp_struct : Inport  Port=3
  nextWp_struct : Inport  Port=4
  preWp_struct : Inport  Port=5
  curPosNEU_m_f : Inport  Port=6
  nav_struct : Inport  Port=7
  perfParams_struct : Inport  Port=8
  ArrivalJudgeSelect : Stateflow chart  TreatAsAtomicUnit=on
  Constant : Constant  Value=false  OutDataTypeStr=boolean
  Constant2 : Constant  Value=false  OutDataTypeStr=boolean
  Multiport Switch : MultiPortSwitch  Inputs=5  DataPortForDefault=Additional data port  DiagnosticForDefault=None  SaturateOnIntegerOverflow=off  InputSameDT=off
  Multiport Switch1 : MultiPortSwitch  Inputs=5  DataPortForDefault=Additional data port  DiagnosticForDefault=None  SaturateOnIntegerOverflow=off  InputSameDT=off
  cirJudge : Subsystem
  fwLineJudge : Subsystem
  hoverPosJudge : Subsystem
  hoverYawJudge : Subsystem
  mcLineJudge : Subsystem
  wpComplete_b : Outport
  isHoverPosReach_b : Outport  Port=2
  wires:
  Multiport Switch/1 -> wpComplete_b/1
  Constant/1 -> Multiport Switch/7
  mssnType_u8/1 -> [mssnType_u8]
  [mssnType_u8] -> ArrivalJudgeSelect/2(mssnType_u8)
  ArrivalJudgeSelect/1(judgeMethod_u8) -> [judgeMethod_u8]
  [judgeMethod_u8] -> Multiport Switch/1
  [judgeMethod_u8] -> Multiport Switch1/1
  ArrivalJudgeSelect/2(hoverPosJudgeEn_b) -> [hoverPosJudgeEn_b]
  ArrivalJudgeSelect/3(hoverYawJudgeEn_b) -> [hoverYawJudgeEn_b]
  ArrivalJudgeSelect/4(mcLineJudgeEn_b) -> [mcLineJudgeEn_b]
  ArrivalJudgeSelect/6(cirJudgeEn_b) -> [cirJudgeEn_b]
  ArrivalJudgeSelect/5(fwLineJudgeEn_b) -> [fwLineJudgeEn_b]
  [hoverPosJudgeEn_b] -> hoverPosJudge/Enable
  [hoverYawJudgeEn_b] -> hoverYawJudge/Enable
  [mcLineJudgeEn_b] -> mcLineJudge/Enable
  [fwLineJudgeEn_b] -> fwLineJudge/Enable
  [cirJudgeEn_b] -> cirJudge/Enable
  hoverPosJudge/1(hoverPosJudge_b) -> [hoverPosJudge_b]
  hoverYawJudge/1(hoverYawJudge_b) -> [hoverYawJudge_b]
  mcLineJudge/1(mcLineJudge_b) -> [mcLineJudge_b]
  fwLineJudge/1(fwLineJudge_b) -> [fwLineJudge_b]
  cirJudge/1(cirJudge_b) -> [cirJudge_b]
  [hoverPosJudge_b] -> Multiport Switch/2
  [hoverYawJudge_b] -> Multiport Switch/3
  [mcLineJudge_b] -> Multiport Switch/4
  [fwLineJudge_b] -> Multiport Switch/5
  [cirJudge_b] -> Multiport Switch/6
  hoverYawJudge/2(isHoverPosReach_b) -> [isHoverPosReach_b]
  [segSwitch_b] -> ArrivalJudgeSelect/3(segSwitch_b)
  segSwitch_b/1 -> [segSwitch_b]
  curWp_struct/1 -> [curWp_struct]
  nextWp_struct/1 -> [nextWp_struct]
  [curWp_struct] -> ArrivalJudgeSelect/1(curWp_struct)
  [nextWp_struct] -> ArrivalJudgeSelect/4(nextWp_struct)
  [preWp_struct] -> ArrivalJudgeSelect/5(preWp_struct)
  preWp_struct/1 -> [preWp_struct]
  Multiport Switch1/1 -> isHoverPosReach_b/1
  Constant2/1 -> Multiport Switch1/6, Multiport Switch1/5, Multiport Switch1/2, Multiport Switch1/4, Multiport Switch1/7
  [isHoverPosReach_b] -> Multiport Switch1/3
  curPosNEU_m_f/1 -> [curPosNEU_m_f]
  [curPosNEU_m_f] -> hoverPosJudge/1(curPosNEU_m_f)
  [curWp_struct] -> hoverPosJudge/2(curWp_struct)
  nav_struct/1 -> [nav_struct]
  [nav_struct] -> hoverPosJudge/3(nav_struct)
  [segSwitch_b] -> hoverPosJudge/4(reset)
  [curPosNEU_m_f] -> hoverYawJudge/1(curPosNEU_m_f)
  [curWp_struct] -> hoverYawJudge/2(curWp_struct)
  [nav_struct] -> hoverYawJudge/3(nav_struct)
  [segSwitch_b] -> hoverYawJudge/4(reset)
  [nextWp_struct] -> hoverYawJudge/5(nextWp_struct)
  [segSwitch_b] -> mcLineJudge/2(reset_b)
  [curPosNEU_m_f] -> mcLineJudge/1(curPosNEU_m_f)
  [preWp_struct] -> mcLineJudge/3(preWp_struct)
  [curWp_struct] -> mcLineJudge/4(curWp_struct)
  [nextWp_struct] -> mcLineJudge/5(nextWp_struct)
  perfParams_struct/1 -> [perfParams_struct]
  [perfParams_struct] -> mcLineJudge/6(perfParams_struct)
  [curPosNEU_m_f] -> fwLineJudge/1(curPosNEU_m_f)
  [segSwitch_b] -> fwLineJudge/2(reset_b)
  [preWp_struct] -> fwLineJudge/3(preWp_struct)
  [curWp_struct] -> fwLineJudge/4(curWp_struct)
  [nextWp_struct] -> fwLineJudge/5(nextWp_struct)
  [segSwitch_b] -> cirJudge/4(reset_b)
  [nextWp_struct] -> cirJudge/3(nextWp_struct)
  [curWp_struct] -> cirJudge/2(curWp_struct)
  [curPosNEU_m_f] -> cirJudge/1(curPosNEU_m_f)

== system GuidanceLaw/Subsystem/wpMssnHandle/WpUpdate ==
  routeUpdate_b : Inport
  wpCompletePulse_b : Inport  Port=2
  validWpNum_u8 : Inport  Port=3
  route_struct : Inport  Port=4
  WaypointManager : Stateflow chart  TreatAsAtomicUnit=on
  WaypointSelector : MATLAB Function  TreatAsAtomicUnit=on
  segSwitch_b : Outport
  routeActive_b : Outport  Port=2
  routeComplete_b : Outport  Port=3
  preWpGeo_struct : Outport  Port=4
  curWpGeo_struct : Outport  Port=5
  nextWpGeo_struct : Outport  Port=6
  wires:
  routeUpdate_b/1 -> [routeUpdate_b]
  [routeUpdate_b] -> WaypointManager/1(routeUpdate_b)
  wpCompletePulse_b/1 -> [wpCompletePulse_b]
  [wpCompletePulse_b] -> WaypointManager/2(wpCompletePulse_b)
  [validWpNum_u8] -> WaypointManager/3(validWpNum_u8)
  validWpNum_u8/1 -> [validWpNum_u8]
  [validWpNum_u8] -> WaypointSelector/2(validWpNum_u8)
  route_struct/1 -> [route_struct]
  [route_struct] -> WaypointSelector/1(route_struct)
  WaypointManager/1(curWpIdx_u8) -> WaypointSelector/3(curWpIdx_u8)
  WaypointManager/2(segSwitch_b) -> segSwitch_b/1
  WaypointManager/3(routeActive_b) -> routeActive_b/1
  WaypointSelector/1(preWp_struct) -> preWpGeo_struct/1
  WaypointSelector/2(curWp_struct) -> curWpGeo_struct/1
  WaypointSelector/3(nextWp_struct) -> nextWpGeo_struct/1
  WaypointManager/4(routeComplete_b) -> routeComplete_b/1
  [route_struct] -> WaypointManager/4(route_struct)

== system GuidanceLaw/Subsystem/wpMssnHandle/GuiLaw/L1CirleGuidance ==
  curPosNE_mps_f : Inport
  nav_struct : Inport  Port=2
  curWp_struct : Inport  Port=3
  reset_b : Inport  Port=4
  perfParams_struct : Inport  Port=5
  Enable : EnablePort  StatesWhenEnabling=reset
  Bus Selector : BusSelector  OutputSignals=pitch_deg_f,yaw_deg_f,velN_mps_f,velE_mps_f,roll_deg_f
  Bus Selector1 : BusSelector  OutputSignals=posN_m_f,posE_m_f,radius_m_f
  Constant : Constant  Value=apParams.G_mps2_f  OutDataTypeStr=single
  Constant1 : Constant  Value=apParams.l1GuiParams.kdCir_f  OutDataTypeStr=single
  Constant2 : Constant  Value=apParams.l1GuiParams.ktCir_f  OutDataTypeStr=single
  Constant3 : Constant  Value=apParams.l1GuiParams.minVxySpd  OutDataTypeStr=single
  Constant4 : Constant  Value=apParams.l1GuiParams.minCirRadius_m_f  OutDataTypeStr=single
  L1CirleGuidance : MATLAB Function  TreatAsAtomicUnit=on
  Vector Concatenate : Concatenate
  rollCmdLimit : Subsystem
  rollCmdLimit_deg_f : Outport
  wires:
  [curPosN_m_f] -> L1CirleGuidance/8(curGpPosN_m_f)
  Constant3/1 -> L1CirleGuidance/5(velXY_min)
  Constant/1 -> L1CirleGuidance/6(G_mps2_f)
  Constant1/1 -> L1CirleGuidance/1(kdCir_f)
  [curVelNE_mps_f] -> L1CirleGuidance/3(curVelNE_mps_f)
  curPosNE_mps_f/1 -> L1CirleGuidance/4(curPosNE_mps_f)
  Constant2/1 -> L1CirleGuidance/2(ktCir_f)
  Constant4/1 -> L1CirleGuidance/11(circle_radius_min)
  [curPosE_m_f] -> L1CirleGuidance/9(curWpPosE_m_f)
  [curYaw_deg_f] -> L1CirleGuidance/12(curYaw_deg_f)
  [curRadius_m_f] -> L1CirleGuidance/10(curWpRadius_m_f)
  [curPitch_deg_f] -> L1CirleGuidance/7(curPitch_deg_f)
  nav_struct/1 -> Bus Selector/1
  Bus Selector/4 -> Vector Concatenate/2  "<velE_mps_f>"
  Bus Selector/2 -> [curYaw_deg_f]  "<yaw_deg_f>"
  Bus Selector/1 -> [curPitch_deg_f]  "<pitch_deg_f>"
  Bus Selector/3 -> Vector Concatenate/1  "<velN_mps_f>"
  Vector Concatenate/1 -> [curVelNE_mps_f]
  Bus Selector1/1 -> [curPosN_m_f]  "<posN_m_f>"
  curWp_struct/1 -> Bus Selector1/1
  Bus Selector1/2 -> [curPosE_m_f]  "<posE_m_f>"
  Bus Selector1/3 -> [curRadius_m_f]  "<radius_m_f>"
  [reset_b] -> rollCmdLimit/4(reset_b)
  L1CirleGuidance/1(rollCmd_deg_f) -> rollCmdLimit/1(rollCmd_mps_f)
  [perfParams_struct] -> rollCmdLimit/2(perfParams_struct)
  [curRoll_deg_f] -> rollCmdLimit/3(curRoll_deg_f)
  rollCmdLimit/1(rollCmdLimit_deg_f) -> rollCmdLimit_deg_f/1
  reset_b/1 -> [reset_b]
  Bus Selector/5 -> [curRoll_deg_f]  "<roll_deg_f>"
  perfParams_struct/1 -> [perfParams_struct]

== system GuidanceLaw/Subsystem/wpMssnHandle/GuiLaw/L1LineGuidance ==
  curPosNE_m_f : Inport
  nav_struct : Inport  Port=2
  mssnType_u8 : Inport  Port=3
  preWp_struct : Inport  Port=4
  curWp_struct : Inport  Port=5
  reset_b : Inport  Port=6
  perfParams_struct : Inport  Port=7
  Enable : EnablePort  StatesWhenEnabling=reset
  Bus Selector : BusSelector  OutputSignals=pitch_deg_f,yaw_deg_f,velN_mps_f,velE_mps_f,roll_deg_f
  Bus Selector1 : BusSelector  OutputSignals=posN_m_f,posE_m_f
  Bus Selector2 : BusSelector  OutputSignals=posN_m_f,posE_m_f
  Constant : Constant  Value=apParams.G_mps2_f  OutDataTypeStr=single
  Constant1 : Constant  Value=apParams.l1GuiParams.kdLine_f  OutDataTypeStr=single
  Constant2 : Constant  Value=apParams.l1GuiParams.ktLine_f  OutDataTypeStr=single
  Constant3 : Constant  Value=apParams.l1GuiParams.minVxySpd  OutDataTypeStr=single
  L1LineGuidance : MATLAB Function  TreatAsAtomicUnit=on
  Vector Concatenate : Concatenate
  rollCmdLimit : Subsystem
  rollCmdLimit_deg_f : Outport
  wires:
  Bus Selector1/1 -> L1LineGuidance/8(curGpPosN_m_f)  "<posN_m_f>"
  Bus Selector2/1 -> L1LineGuidance/10(preGpPosN_m_f)  "<posN_m_f>"
  Bus Selector2/2 -> L1LineGuidance/11(preGpPosE_m_f)  "<posE_m_f>"
  Bus Selector1/2 -> L1LineGuidance/9(curGpPosE_m_f)  "<posE_m_f>"
  [curYaw_deg_f] -> L1LineGuidance/13(curYaw_deg_f)
  [mssnType_u8] -> L1LineGuidance/12(mssnType_u8)
  L1LineGuidance/1(rollCmd_deg_f) -> rollCmdLimit/1(rollCmd_mps_f)
  Constant1/1 -> L1LineGuidance/1(kdLine_f)
  [curVelNE_mps_f] -> L1LineGuidance/3(curVelNE_mps_f)
  Constant2/1 -> L1LineGuidance/2(ktLine_f)
  [curPitch_deg_f] -> L1LineGuidance/7(curPitch_deg_f)
  curPosNE_m_f/1 -> L1LineGuidance/4(curPosNE_m_f)
  Constant3/1 -> L1LineGuidance/5(velXY_min)
  Constant/1 -> L1LineGuidance/6(G_mps2_f)
  mssnType_u8/1 -> [mssnType_u8]
  nav_struct/1 -> Bus Selector/1
  Bus Selector/1 -> [curPitch_deg_f]  "<pitch_deg_f>"
  Bus Selector/2 -> [curYaw_deg_f]  "<yaw_deg_f>"
  Bus Selector/3 -> Vector Concatenate/1  "<velN_mps_f>"
  Bus Selector/4 -> Vector Concatenate/2  "<velE_mps_f>"
  Vector Concatenate/1 -> [curVelNE_mps_f]
  preWp_struct/1 -> [preWp_struct]
  curWp_struct/1 -> [curWp_struct]
  [curWp_struct] -> Bus Selector1/1
  [preWp_struct] -> Bus Selector2/1
  rollCmdLimit/1(rollCmdLimit_deg_f) -> rollCmdLimit_deg_f/1
  reset_b/1 -> [reset_b]
  [reset_b] -> rollCmdLimit/4(reset_b)
  Bus Selector/5 -> [curRoll_deg_f]  "<roll_deg_f>"
  [curRoll_deg_f] -> rollCmdLimit/3(curRoll_deg_f)
  perfParams_struct/1 -> [perfParams_struct]
  [perfParams_struct] -> rollCmdLimit/2(perfParams_struct)

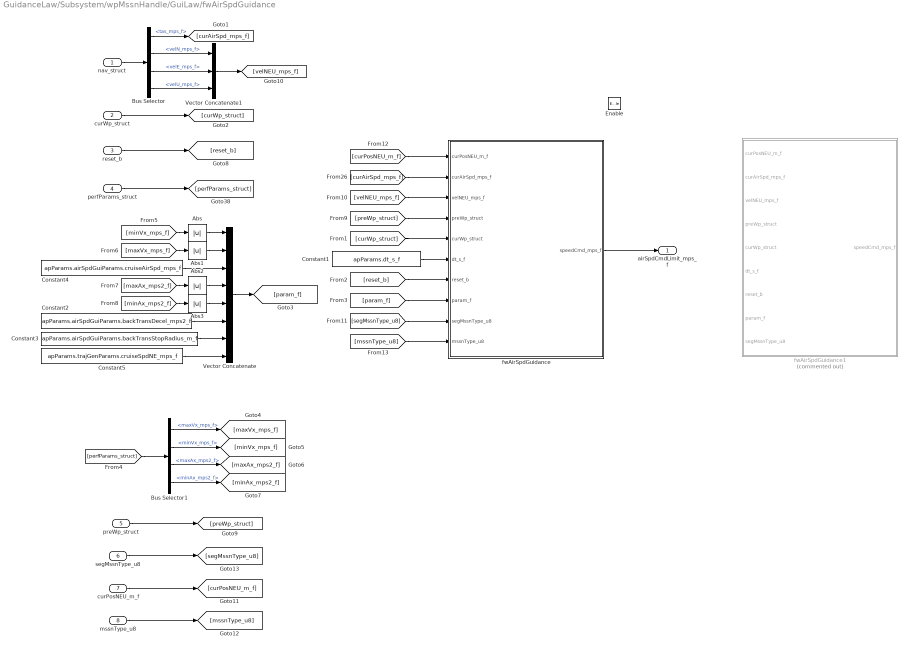
== system GuidanceLaw/Subsystem/wpMssnHandle/GuiLaw/fwAirSpdGuidance ==
  nav_struct : Inport
  curWp_struct : Inport  Port=2
  reset_b : Inport  Port=3
  perfParams_struct : Inport  Port=4
  preWp_struct : Inport  Port=5
  segMssnType_u8 : Inport  Port=6
  curPosNEU_m_f : Inport  Port=7
  mssnType_u8 : Inport  Port=8
  Enable : EnablePort  StatesWhenEnabling=reset
  Abs{,1..3} (4 alike) : Abs  SaturateOnIntegerOverflow=off
  Bus Selector : BusSelector  OutputSignals=tas_mps_f,velN_mps_f,velE_mps_f,velU_mps_f
  Bus Selector1 : BusSelector  OutputSignals=maxVx_mps_f,minVx_mps_f,maxAx_mps2_f,minAx_mps2_f
  Constant1 : Constant  Value=apParams.dt_s_f  OutDataTypeStr=single
  Constant2 : Constant  Value=apParams.airSpdGuiParams.backTransDecel_mps2_f  OutDataTypeStr=single
  Constant3 : Constant  Value=apParams.airSpdGuiParams.backTransStopRadius_m_f  OutDataTypeStr=single
  Constant4 : Constant  Value=apParams.airSpdGuiParams.cruiseAirSpd_mps_f  OutDataTypeStr=single
  Constant5 : Constant  Value=apParams.trajGenParams.cruiseSpdNE_mps_f  OutDataTypeStr=single
  Vector Concatenate : Concatenate  NumInputs=8
  Vector Concatenate1 : Concatenate  NumInputs=3
  fwAirSpdGuidance : MATLAB Function  TreatAsAtomicUnit=on
  fwAirSpdGuidance1 : MATLAB Function  Commented=on  TreatAsAtomicUnit=on
  airSpdCmdLimit_mps_f : Outport
  wires:
  nav_struct/1 -> Bus Selector/1
  Bus Selector/1 -> [curAirSpd_mps_f]  "<tas_mps_f>"
  [curAirSpd_mps_f] -> fwAirSpdGuidance/2(curAirSpd_mps_f)
  curWp_struct/1 -> [curWp_struct]
  [curWp_struct] -> fwAirSpdGuidance/5(curWp_struct)
  Constant1/1 -> fwAirSpdGuidance/6(dt_s_f)
  reset_b/1 -> [reset_b]
  [reset_b] -> fwAirSpdGuidance/7(reset_b)
  Vector Concatenate/1 -> [param_f]
  Constant4/1 -> Vector Concatenate/3
  [maxAx_mps2_f] -> Abs2/1
  [minAx_mps2_f] -> Abs3/1
  [param_f] -> fwAirSpdGuidance/8(param_f)
  [minVx_mps_f] -> Abs/1
  [maxVx_mps_f] -> Abs1/1
  perfParams_struct/1 -> [perfParams_struct]
  [perfParams_struct] -> Bus Selector1/1
  Bus Selector1/1 -> [maxVx_mps_f]  "<maxVx_mps_f>"
  Bus Selector1/2 -> [minVx_mps_f]  "<minVx_mps_f>"
  Bus Selector1/3 -> [maxAx_mps2_f]  "<maxAx_mps2_f>"
  Bus Selector1/4 -> [minAx_mps2_f]  "<minAx_mps2_f>"
  preWp_struct/1 -> [preWp_struct]
  [preWp_struct] -> fwAirSpdGuidance/4(preWp_struct)
  [velNEU_mps_f] -> fwAirSpdGuidance/3(velNEU_mps_f)
  Bus Selector/2 -> Vector Concatenate1/1  "<velN_mps_f>"
  Bus Selector/3 -> Vector Concatenate1/2  "<velE_mps_f>"
  Bus Selector/4 -> Vector Concatenate1/3  "<velU_mps_f>"
  Vector Concatenate1/1 -> [velNEU_mps_f]
  Constant2/1 -> Vector Concatenate/6
  Constant3/1 -> Vector Concatenate/7
  Abs/1 -> Vector Concatenate/1
  Abs1/1 -> Vector Concatenate/2
  Abs2/1 -> Vector Concatenate/4
  Abs3/1 -> Vector Concatenate/5
  fwAirSpdGuidance/1(speedCmd_mps_f) -> airSpdCmdLimit_mps_f/1
  segMssnType_u8/1 -> [segMssnType_u8]
  [segMssnType_u8] -> fwAirSpdGuidance/9(segMssnType_u8)
  [curPosNEU_m_f] -> fwAirSpdGuidance/1(curPosNEU_m_f)
  curPosNEU_m_f/1 -> [curPosNEU_m_f]
  Constant5/1 -> Vector Concatenate/8
  mssnType_u8/1 -> [mssnType_u8]
  [mssnType_u8] -> fwAirSpdGuidance/10(mssnType_u8)
